simulink model "VCU_2023"  (Simulink 10.1)
settings: Solver=FixedStepDiscrete  StartTime=0.0  StopTime=10.0  FixedStep=0.001  RelTol=1e-3  EnableMultiTasking=on
PreLoadFcn:
  | try
  | MDL_setup;
  | catch
  | end
InitFcn:
  | EcoCoder_PreCheckLic();
undefined symbols (not defined in the file): APPS1_max, APPS1_min, APPS2_max, APPS2_min, BRK_TH, DiscIntNeverNeededParam, sigbuilder_block
libraries: CoderSF_BSW_Libs x188, simulink x28
(part 3 of 3)

== system VCU_2023/Main/CANbus Management/Asking data from the inverter/Value separation/I_nom_eff ==
  Time interval : Inport
  Trigger : TriggerPort  VariantControl=Variant
  Constant : Constant  Value=hex2dec('3d')  OutDataTypeStr=uint8
  Constant1 : Constant  Value=hex2dec('4e')  OutDataTypeStr=uint8
  Pack Signals To CAN Data : CoderSF_BSW_Libs/CAN/Pack Signals To CAN Data  Signal="{{'REG_31'  'Data1' 'Data2'},[0 8 16],[8 8 8],{'uint8'  'uint8' 'uint8'},{'Intel' 'Intel' 'Intel'}}"
  Send CAN Data : CoderSF_BSW_Libs/CAN/Send CAN Data  channel=CAN_A  txlen=3  txid=hex2dec('201')  frametype=Standard(11-bit ID)  showerror=off
  wires:
  Constant/1 -> Pack Signals To CAN Data/1
  Pack Signals To CAN Data/1 -> Send CAN Data/1
  Constant1/1 -> Pack Signals To CAN Data/2
  Time interval/1 -> Pack Signals To CAN Data/3

== system VCU_2023/Main/CANbus Management/Asking data from the inverter/Value separation/N_100 ==
  Time interval : Inport
  Trigger : TriggerPort  VariantControl=Variant
  Constant : Constant  Value=hex2dec('3d')  OutDataTypeStr=uint8
  Constant1 : Constant  Value=hex2dec('c8')  OutDataTypeStr=uint8
  Pack Signals To CAN Data : CoderSF_BSW_Libs/CAN/Pack Signals To CAN Data  Signal="{{'REG_31'  'Data1' 'Data2'},[0 8 16],[8 8 8],{'uint8'  'uint8' 'uint8'},{'Intel' 'Intel' 'Intel'}}"
  Send CAN Data : CoderSF_BSW_Libs/CAN/Send CAN Data  channel=CAN_A  txlen=3  txid=hex2dec('201')  frametype=Standard(11-bit ID)  showerror=off
  wires:
  Constant/1 -> Pack Signals To CAN Data/1
  Pack Signals To CAN Data/1 -> Send CAN Data/1
  Constant1/1 -> Pack Signals To CAN Data/2
  Time interval/1 -> Pack Signals To CAN Data/3

== system VCU_2023/Main/CANbus Management/Asking data from the inverter/Value separation/N_Lim ==
  Time interval : Inport
  Trigger : TriggerPort  VariantControl=Variant
  Constant : Constant  Value=hex2dec('3d')  OutDataTypeStr=uint8
  Constant1 : Constant  Value=hex2dec('34')  OutDataTypeStr=uint8
  Pack Signals To CAN Data : CoderSF_BSW_Libs/CAN/Pack Signals To CAN Data  Signal="{{'REG_31'  'Data1' 'Data2'},[0 8 16],[8 8 8],{'uint8'  'uint8' 'uint8'},{'Intel' 'Intel' 'Intel'}}"
  Send CAN Data : CoderSF_BSW_Libs/CAN/Send CAN Data  channel=CAN_A  txlen=3  txid=hex2dec('201')  frametype=Standard(11-bit ID)  showerror=off
  wires:
  Constant/1 -> Pack Signals To CAN Data/1
  Pack Signals To CAN Data/1 -> Send CAN Data/1
  Constant1/1 -> Pack Signals To CAN Data/2
  Time interval/1 -> Pack Signals To CAN Data/3

== system VCU_2023/Main/CANbus Management/Asking data from the inverter/Value separation/N_Lim_neg ==
  Time interval : Inport
  Trigger : TriggerPort  VariantControl=Variant
  Constant : Constant  Value=hex2dec('3d')  OutDataTypeStr=uint8
  Constant1 : Constant  Value=hex2dec('3e')  OutDataTypeStr=uint8
  Pack Signals To CAN Data : CoderSF_BSW_Libs/CAN/Pack Signals To CAN Data  Signal="{{'REG_31'  'Data1' 'Data2'},[0 8 16],[8 8 8],{'uint8'  'uint8' 'uint8'},{'Intel' 'Intel' 'Intel'}}"
  Send CAN Data : CoderSF_BSW_Libs/CAN/Send CAN Data  channel=CAN_A  txlen=3  txid=hex2dec('201')  frametype=Standard(11-bit ID)  showerror=off
  wires:
  Constant/1 -> Pack Signals To CAN Data/1
  Pack Signals To CAN Data/1 -> Send CAN Data/1
  Constant1/1 -> Pack Signals To CAN Data/2
  Time interval/1 -> Pack Signals To CAN Data/3

== system VCU_2023/Main/CANbus Management/Asking data from the inverter/Value separation/N_Lim_pos ==
  Time interval : Inport
  Trigger : TriggerPort  VariantControl=Variant
  Constant : Constant  Value=hex2dec('3d')  OutDataTypeStr=uint8
  Constant1 : Constant  Value=hex2dec('3f')  OutDataTypeStr=uint8
  Pack Signals To CAN Data : CoderSF_BSW_Libs/CAN/Pack Signals To CAN Data  Signal="{{'REG_31'  'Data1' 'Data2'},[0 8 16],[8 8 8],{'uint8'  'uint8' 'uint8'},{'Intel' 'Intel' 'Intel'}}"
  Send CAN Data : CoderSF_BSW_Libs/CAN/Send CAN Data  channel=CAN_A  txlen=3  txid=hex2dec('201')  frametype=Standard(11-bit ID)  showerror=off
  wires:
  Constant/1 -> Pack Signals To CAN Data/1
  Pack Signals To CAN Data/1 -> Send CAN Data/1
  Constant1/1 -> Pack Signals To CAN Data/2
  Time interval/1 -> Pack Signals To CAN Data/3

== system VCU_2023/Main/CANbus Management/Asking data from the inverter/Value separation/N_R_Acc | M_R_Acc ==
  Time interval : Inport
  Trigger : TriggerPort  VariantControl=Variant
  Constant : Constant  Value=hex2dec('3d')  OutDataTypeStr=uint8
  Constant1 : Constant  Value=hex2dec('35')  OutDataTypeStr=uint8
  Pack Signals To CAN Data : CoderSF_BSW_Libs/CAN/Pack Signals To CAN Data  Signal="{{'REG_31'  'Data1' 'Data2'},[0 8 16],[8 8 8],{'uint8'  'uint8' 'uint8'},{'Intel' 'Intel' 'Intel'}}"
  Send CAN Data : CoderSF_BSW_Libs/CAN/Send CAN Data  channel=CAN_A  txlen=3  txid=hex2dec('201')  frametype=Standard(11-bit ID)  showerror=off
  wires:
  Constant/1 -> Pack Signals To CAN Data/1
  Pack Signals To CAN Data/1 -> Send CAN Data/1
  Constant1/1 -> Pack Signals To CAN Data/2
  Time interval/1 -> Pack Signals To CAN Data/3

== system VCU_2023/Main/CANbus Management/Asking data from the inverter/Value separation/N_R_Dec | M_R_Dec ==
  Time interval : Inport
  Trigger : TriggerPort  VariantControl=Variant
  Constant : Constant  Value=hex2dec('3d')  OutDataTypeStr=uint8
  Constant1 : Constant  Value=hex2dec('ed')  OutDataTypeStr=uint8
  Pack Signals To CAN Data : CoderSF_BSW_Libs/CAN/Pack Signals To CAN Data  Signal="{{'REG_31'  'Data1' 'Data2'},[0 8 16],[8 8 8],{'uint8'  'uint8' 'uint8'},{'Intel' 'Intel' 'Intel'}}"
  Send CAN Data : CoderSF_BSW_Libs/CAN/Send CAN Data  channel=CAN_A  txlen=3  txid=hex2dec('201')  frametype=Standard(11-bit ID)  showerror=off
  wires:
  Constant/1 -> Pack Signals To CAN Data/1
  Pack Signals To CAN Data/1 -> Send CAN Data/1
  Constant1/1 -> Pack Signals To CAN Data/2
  Time interval/1 -> Pack Signals To CAN Data/3

== system VCU_2023/Main/CANbus Management/Asking data from the inverter/Value separation/Repeatedly asked values ==
  note: These values will be sent every 100ms
  Trigger : TriggerPort  VariantControl=Variant
  Constant1 : Constant  Value=hex2dec('64')  OutDataTypeStr=uint8
  I_act_filt : Subsystem
  I_cmd : Subsystem
  N_act_filt : Subsystem
  T_IGBT : Subsystem
  T_air : Subsystem
  T_motor : Subsystem
  Vdc_bus : Subsystem
  wires:
  Constant1/1 -> T_air/1(Time interval), T_motor/1(Time interval), T_IGBT/1(Time interval), I_cmd/1(Time interval), I_act_filt/1(Time interval), Vdc_bus/1(Time interval), N_act_filt/1(Time interval)

== system VCU_2023/Main/CANbus Management/Asking data from the inverter/Value separation/SpeedRPMmax ==
  Time interval : Inport
  Trigger : TriggerPort  VariantControl=Variant
  Constant : Constant  Value=hex2dec('3d')  OutDataTypeStr=uint8
  Constant1 : Constant  Value=hex2dec('ce')  OutDataTypeStr=uint8
  Pack Signals To CAN Data : CoderSF_BSW_Libs/CAN/Pack Signals To CAN Data  Signal="{{'REG_31'  'Data1' 'Data2'},[0 8 16],[8 8 8],{'uint8'  'uint8' 'uint8'},{'Intel' 'Intel' 'Intel'}}"
  Send CAN Data : CoderSF_BSW_Libs/CAN/Send CAN Data  channel=CAN_A  txlen=3  txid=hex2dec('201')  frametype=Standard(11-bit ID)  showerror=off
  wires:
  Constant/1 -> Pack Signals To CAN Data/1
  Pack Signals To CAN Data/1 -> Send CAN Data/1
  Constant1/1 -> Pack Signals To CAN Data/2
  Time interval/1 -> Pack Signals To CAN Data/3

== system VCU_2023/Main/Main Functionalities/Ready to drive/Subsystem1/Enter R2D Mode ==
  Exit : Inport
  Trigger : TriggerPort  VariantControl=Variant  OutputDataType=int8  InitialTriggerSignalState=zero
  Constant1 : Constant  OutDataTypeStr=boolean
  Constant2 : Constant  OutDataTypeStr=boolean
  Logical Operator2 : Logic  IconShape=distinctive  AllPortsSameDT=off  OutDataTypeStr=boolean
  Logical Operator3 : Logic  IconShape=distinctive  AllPortsSameDT=off  OutDataTypeStr=boolean
  R2D Sound : Outport
  R2D Led : Outport  Port=2
  wires:
  Exit/1 -> Logical Operator3/1, Logical Operator2/2
  Logical Operator2/1 -> R2D Led/1
  Constant1/1 -> Logical Operator2/1
  Logical Operator3/1 -> R2D Sound/1
  Constant2/1 -> Logical Operator3/2

== system VCU_2023/Main/Main Functionalities/Tractive System/Subsystem/Subsystem ==
  In1 : Inport
  Trigger : TriggerPort  VariantControl=Variant  PortDimensions=1
  Logical Operator : Logic  AllPortsSameDT=off  OutDataTypeStr=boolean
  Logical Operator1 : Logic  Operator=NOT  IconShape=distinctive  AllPortsSameDT=off  OutDataTypeStr=boolean
  Read NVM : CoderSF_BSW_Libs/Non-volatile Memory Blocks/Read NVM  variable_name=nvm_TS_ON  variable_type=Inherit from 'Variable definition'
  TS ON : Outport
  wires:
  Logical Operator1/1 -> Logical Operator/1
  In1/1 -> Logical Operator/2
  Read NVM/1 -> Logical Operator1/1
  Logical Operator/1 -> TS ON/1

== system VCU_2023/Main/CANbus Management/Asking data from the inverter/Value separation/Repeatedly asked values/I_act_filt ==
  Time interval : Inport
  Constant : Constant  Value=hex2dec('3d')  OutDataTypeStr=uint8
  Constant1 : Constant  Value=hex2dec('5f')  OutDataTypeStr=uint8
  Pack Signals To CAN Data : CoderSF_BSW_Libs/CAN/Pack Signals To CAN Data  Signal="{{'REG_31'  'Data1' 'Data2'},[0 8 16],[8 8 8],{'uint8'  'uint8' 'uint8'},{'Intel' 'Intel' 'Intel'}}"
  Send CAN Data : CoderSF_BSW_Libs/CAN/Send CAN Data  channel=CAN_A  txlen=3  txid=hex2dec('201')  frametype=Standard(11-bit ID)  showerror=off
  wires:
  Constant/1 -> Pack Signals To CAN Data/1
  Pack Signals To CAN Data/1 -> Send CAN Data/1
  Constant1/1 -> Pack Signals To CAN Data/2
  Time interval/1 -> Pack Signals To CAN Data/3

== system VCU_2023/Main/CANbus Management/Asking data from the inverter/Value separation/Repeatedly asked values/I_cmd ==
  Time interval : Inport
  Constant : Constant  Value=hex2dec('3d')  OutDataTypeStr=uint8
  Constant1 : Constant  Value=hex2dec('26')  OutDataTypeStr=uint8
  Pack Signals To CAN Data : CoderSF_BSW_Libs/CAN/Pack Signals To CAN Data  Signal="{{'REG_31'  'Data1' 'Data2'},[0 8 16],[8 8 8],{'uint8'  'uint8' 'uint8'},{'Intel' 'Intel' 'Intel'}}"
  Send CAN Data : CoderSF_BSW_Libs/CAN/Send CAN Data  channel=CAN_A  txlen=3  txid=hex2dec('201')  frametype=Standard(11-bit ID)  showerror=off
  wires:
  Constant/1 -> Pack Signals To CAN Data/1
  Pack Signals To CAN Data/1 -> Send CAN Data/1
  Constant1/1 -> Pack Signals To CAN Data/2
  Time interval/1 -> Pack Signals To CAN Data/3

== system VCU_2023/Main/CANbus Management/Asking data from the inverter/Value separation/Repeatedly asked values/N_act_filt ==
  Time interval : Inport
  Constant : Constant  Value=hex2dec('3d')  OutDataTypeStr=uint8
  Constant1 : Constant  Value=hex2dec('a8')  OutDataTypeStr=uint8
  Pack Signals To CAN Data : CoderSF_BSW_Libs/CAN/Pack Signals To CAN Data  Signal="{{'REG_31'  'Data1' 'Data2'},[0 8 16],[8 8 8],{'uint8'  'uint8' 'uint8'},{'Intel' 'Intel' 'Intel'}}"
  Send CAN Data : CoderSF_BSW_Libs/CAN/Send CAN Data  channel=CAN_A  txlen=3  txid=hex2dec('201')  frametype=Standard(11-bit ID)  showerror=off
  wires:
  Constant/1 -> Pack Signals To CAN Data/1
  Pack Signals To CAN Data/1 -> Send CAN Data/1
  Constant1/1 -> Pack Signals To CAN Data/2
  Time interval/1 -> Pack Signals To CAN Data/3

== system VCU_2023/Main/CANbus Management/Asking data from the inverter/Value separation/Repeatedly asked values/T_IGBT ==
  Time interval : Inport
  Constant : Constant  Value=hex2dec('3d')  OutDataTypeStr=uint8
  Constant1 : Constant  Value=hex2dec('4a')  OutDataTypeStr=uint8
  Pack Signals To CAN Data : CoderSF_BSW_Libs/CAN/Pack Signals To CAN Data  Signal="{{'REG_31'  'Data1' 'Data2'},[0 8 16],[8 8 8],{'uint8'  'uint8' 'uint8'},{'Intel' 'Intel' 'Intel'}}"
  Send CAN Data : CoderSF_BSW_Libs/CAN/Send CAN Data  channel=CAN_A  txlen=3  txid=hex2dec('201')  frametype=Standard(11-bit ID)  showerror=off
  wires:
  Constant/1 -> Pack Signals To CAN Data/1
  Pack Signals To CAN Data/1 -> Send CAN Data/1
  Constant1/1 -> Pack Signals To CAN Data/2
  Time interval/1 -> Pack Signals To CAN Data/3

== system VCU_2023/Main/CANbus Management/Asking data from the inverter/Value separation/Repeatedly asked values/T_air ==
  Time interval : Inport
  Constant : Constant  Value=hex2dec('3d')  OutDataTypeStr=uint8
  Constant1 : Constant  Value=hex2dec('4b')  OutDataTypeStr=uint8
  Pack Signals To CAN Data : CoderSF_BSW_Libs/CAN/Pack Signals To CAN Data  Signal="{{'REG_31'  'Data1' 'Data2'},[0 8 16],[8 8 8],{'uint8'  'uint8' 'uint8'},{'Intel' 'Intel' 'Intel'}}"
  Send CAN Data : CoderSF_BSW_Libs/CAN/Send CAN Data  channel=CAN_A  txlen=3  txid=hex2dec('201')  frametype=Standard(11-bit ID)  showerror=off
  wires:
  Constant/1 -> Pack Signals To CAN Data/1
  Pack Signals To CAN Data/1 -> Send CAN Data/1
  Constant1/1 -> Pack Signals To CAN Data/2
  Time interval/1 -> Pack Signals To CAN Data/3

== system VCU_2023/Main/CANbus Management/Asking data from the inverter/Value separation/Repeatedly asked values/T_motor ==
  Time interval : Inport
  Constant : Constant  Value=hex2dec('3d')  OutDataTypeStr=uint8
  Constant1 : Constant  Value=hex2dec('49')  OutDataTypeStr=uint8
  Pack Signals To CAN Data : CoderSF_BSW_Libs/CAN/Pack Signals To CAN Data  Signal="{{'REG_31'  'Data1' 'Data2'},[0 8 16],[8 8 8],{'uint8'  'uint8' 'uint8'},{'Intel' 'Intel' 'Intel'}}"
  Send CAN Data : CoderSF_BSW_Libs/CAN/Send CAN Data  channel=CAN_A  txlen=3  txid=hex2dec('201')  frametype=Standard(11-bit ID)  showerror=off
  wires:
  Constant/1 -> Pack Signals To CAN Data/1
  Pack Signals To CAN Data/1 -> Send CAN Data/1
  Constant1/1 -> Pack Signals To CAN Data/2
  Time interval/1 -> Pack Signals To CAN Data/3

== system VCU_2023/Main/CANbus Management/Asking data from the inverter/Value separation/Repeatedly asked values/Vdc_bus ==
  Time interval : Inport
  Constant : Constant  Value=hex2dec('3d')  OutDataTypeStr=uint8
  Constant1 : Constant  Value=hex2dec('eb')  OutDataTypeStr=uint8
  Pack Signals To CAN Data : CoderSF_BSW_Libs/CAN/Pack Signals To CAN Data  Signal="{{'REG_31'  'Data1' 'Data2'},[0 8 16],[8 8 8],{'uint8'  'uint8' 'uint8'},{'Intel' 'Intel' 'Intel'}}"
  Send CAN Data : CoderSF_BSW_Libs/CAN/Send CAN Data  channel=CAN_A  txlen=3  txid=hex2dec('201')  frametype=Standard(11-bit ID)  showerror=off
  wires:
  Constant/1 -> Pack Signals To CAN Data/1
  Pack Signals To CAN Data/1 -> Send CAN Data/1
  Constant1/1 -> Pack Signals To CAN Data/2
  Time interval/1 -> Pack Signals To CAN Data/3
